simulink model "SolarPanelValidation"  (R2025a)
settings: Solver=VariableStepAuto  StartTime=0.0  StopTime=1.1*Voc/1  FixedStep=Ts  MaxStep=1e-3  RelTol=1e-3
PreLoadFcn:
  | % Parameterize the panel
  | SolarPanelValidationInput;
  | 
  | % Set the default test condition
  | irradiance = 1000;
  | temperature = 25;
values from neighbouring files (symbols this model uses):
  Isc = 8.18    [SolarPanelValidationInput.m]
  Np_cell = 3    [SolarPanelValidationInput.m]
  Ns_cell = 60    [SolarPanelValidationInput.m]
  Voc = 36.7    [SolarPanelValidationInput.m]
libraries: fl_lib x3, nesl_utility x3, ee_lib x1, simulink x1
CloseFcn:
  | try,close(h1_SolarPanelValidation),end
  | clear h1_SolarPanelValidation
  | 
  | clear CellTemperature  MaximumVoltage    TXIS1  irradianceVec
  | clear Irad NQ Tct  simlog_SolarPanelValidation
  | clear Isc Np_cell Tmeas  temperature
  | clear MaxP Ns_cell Voc  temperatureVec
  | clear MaximumCurrent  tout
  | clear MaximumPower  Rs   irradiance PanelIrradiance
Description:
  | Solar Panel Parameterization Validation
settings Model: Creator=The MathWorks, Inc.  LastModifiedBy=The MathWorks, Inc.
settings SolverCC: InitialStep=1e-3  AlgebraicLoopSolver=TrustRegion
settings DataIOCC: ReturnWorkspaceOutputs=off  OutputOption=SpecifiedOutputTimes  OutputTimes=[0:1.1*Voc/(1*1300):1.1*Voc/1]
settings OptimizationCC: ReuseModelBlockBuffer=off
settings DebuggingCC: UnconnectedInputMsg=warning  UnconnectedOutputMsg=warning  UnconnectedLineMsg=warning  StateNameClashWarn=warning  ArithmeticOperatorsInVariantConditions=warning
settings HardwareCC: ProdBitPerPointer=32.0  ProdBitPerSizeT=32.0  ProdBitPerPtrDiffT=32.0  ProdWordSize=32.0  ProdHWDeviceType=Intel->x86-32 (Windows32)
settings ModelReferenceCC: EnableRefExpFcnMdlSchedulingChecks=on  PropagateSignalLabelsOutOfModel=off
settings SFSimCC: CustomCodeUndefinedFunction=UseInterfaceOnly
settings RTWCC: GPUComputeCapability=3.5  DLArmComputeVersion=19.05
settings CodeAppCC: StateflowObjectComments=on
settings SimscapeCC: SimscapeLogType=all  SimscapeLogSimulationStatistics=on  SimscapeLogName=simlog_SolarPanelValidation

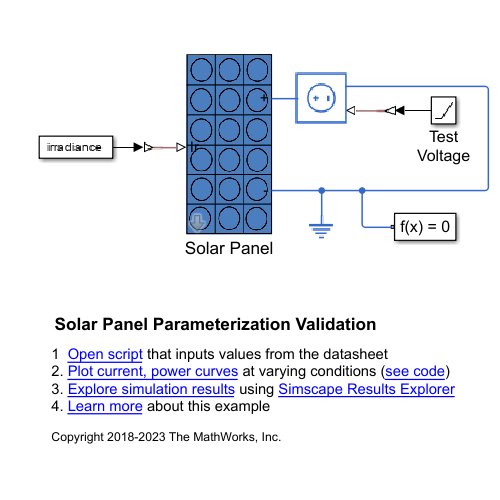
[thumbnail: Simulink's stored preview of the top-level diagram]
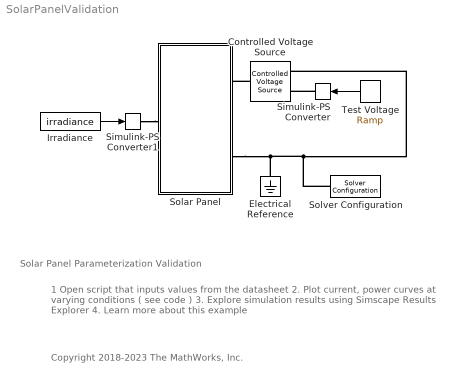
== system SolarPanelValidation ==
  note: Solar Panel Parameterization Validation
  note: 1 Open script that inputs values from the datasheet
      | 2. Plot current, power curves at varying conditions ( see code )
      | 3. Explore simulation results using Simscape Results Explorer
      | 4. Learn more about this example
  note: Copyright 2018-2023 The MathWorks, Inc.
  Controlled Voltage Source : fl_lib/Electrical/Electrical Sources/Controlled Voltage Source
  Electrical Reference : fl_lib/Electrical/Electrical Elements/Electrical Reference
  Irradiance : Constant  Value=irradiance
  Simulink-PS Converter : nesl_utility/Simulink-PS Converter  PhysicalDomain=network_engine_domain  SubClassName=ps_input  LeftPortType=input  RightPortType=output  PseudoPeriodic=off  Frequencies=[]  NoiseDistribution=none  NoiseParameters=[]  Unit=1  AffineConversion=off  FilteringAndDerivatives=provide  SimscapeFilterOrder=1  InputFilterTimeConstant=0.001  UdotUserProvided=0
  Simulink-PS Converter1 : nesl_utility/Simulink-PS Converter  PhysicalDomain=network_engine_domain  SubClassName=ps_input  LeftPortType=input  RightPortType=output  PseudoPeriodic=off  Frequencies=[]  NoiseDistribution=none  NoiseParameters=[]  Unit=1  AffineConversion=off  FilteringAndDerivatives=provide  SimscapeFilterOrder=1  InputFilterTimeConstant=0.001  UdotUserProvided=0
  Solar Panel : Subsystem  mask(Solar Panel){}
      mask help: Models a solar panel using a parallel-connected string of solar cells. The solar cell strings are modeled using a single Solar Cell block from the Simscape(TM) Electrical(TM) Sources library.
      mask Display: image('SolarPanelValidationIcon.jpg')
  Solver Configuration : nesl_utility/Solver Configuration  PhysicalDomain=network_engine_domain  SubClassName=solver  LeftPortType=input  RightPortType=generic  Tones=[]  Harmonics=[]  SimulateNoise=off  Profile=off  UseLocalSampling=off  EnableSwitchedLinearOptims=on  FrequencyDomain=off  UseCCode=off  RelTol=0.001  AbsTol=1e-06  MinStep=1e-09  ToWorkspace=off  RevertToSquareIcSolve=off  NumHomotopyIterations=100  PhasorMode=off  PhasorModeNumHarmonics=1  ConsistencySolver=NEWTON_FTOL  IndexReductionMethod=DerivativeReplacement  DoDC=off  ResidualTolerance=1e-09  ConsistencyTolSource=GLOBAL  ConsistencyAbsTol=0.001  ConsistencyRelTol=0.001  ConsistencyTolFactor=0.001  UseLocalSolver=off  LocalSolverChoice=NE_BACKWARD_EULER_ADVANCER  ResolveIndetEquations=on  FunctionEvalNumThread=1  LocalSolverSampleTime=1e-4  DoFixedCost=off  MaxNonlinIter=3  MaxModeIter=2  ComputeImpulses=off  ImpulseIterations=1  LinearAlgebra=auto  LinearAlgebraNumThread=0  EquationFormulation=NE_TIME_EF  DelaysMemoryBudget=1024  AutomaticFiltering=on  FilteringTimeConstant=0.001  PartitionStorageMethod=AS_NEEDED  PartitionMemoryBudget=1024  PartitionMethod=ROBUST  MultibodyUseLocalSolver=off  MultibodyLocalSolverChoice=ODE1  MultibodyLocalSolverSampleTime=0.001
  Test Voltage : simulink/Sources/Ramp  slope=1  start=0  InitialOutput=0
  wires:
  Irradiance/1 -> Simulink-PS Converter1/1
  Test Voltage/1 -> Simulink-PS Converter/1
  connections:
  Solver Configuration/RConn1 -- Controlled Voltage Source/RConn2 -- Electrical Reference/LConn1 -- Solar Panel/RConn2
  Controlled Voltage Source/LConn1 -- Solar Panel/RConn1
  Simulink-PS Converter/RConn1 -- Controlled Voltage Source/RConn1
  Simulink-PS Converter1/RConn1 -- Solar Panel/LConn1

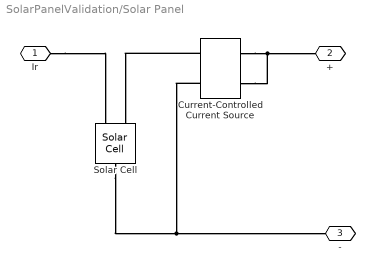
== system SolarPanelValidation/Solar Panel ==
  Current-Controlled Current Source : fl_lib/Electrical/Electrical Sources/Current-Controlled Current Source  K=-1*(Np_cell-1)  i1_specify=off  i1_priority=None  i1=0 A  i1_nominal_specify=off  i1_nominal_value=1  i1_nominal_unit=A  i2_specify=off  i2_priority=None  i2=0 A  i2_nominal_specify=off  i2_nominal_value=1  i2_nominal_unit=A
      settings: InternalSimscapePortConfiguration="{\"Bottom\":[],\"Left\":[{\"id\":\"p1\",\"label\":\"+\",\"type\":\"foundation.electrical.electrical\"},{\"id\":\"head\",\"label\":\"\",\"type\":\"foundation.electrical.electrical\"}],\"Right\":[{\"id\":\"n1\",\"label\":\"-\",\"type\":\"foundation.electrical.electrical\"},{\"id\":\"tail\",\"label\":\"\",\"type\":\"foundation.electrical.electrical\"}],\"Top\":[]}"
  Solar Cell : ee_lib/Sources/Solar Cell  prm=1  Isc=Isc/Np_cell A  Voc=Voc/Ns_cell V  Is=1e-6 A  Is2=0 A  Iph=7.34 A  Ir0=Irad W/m^2  ec=NQ  N2=2  Rs=Rs Ohm  Rp=inf Ohm  N_series=Ns_cell  N_parallel=1  TIPH1=Tct 1/K  EG=1.11 eV  TXIS1=TXIS1  TXIS2=3  TRS1=0  TRP1=0  Tmeas=Tmeas degC  TFIXED=temperature degC  thermal_mass=100 J/K  initial_temperature=25 degC
  Ir : PMIOPort  Side=Left
  + : PMIOPort  Port=2  Side=Right
  - : PMIOPort  Port=3  Side=Right
  connections:
  Current-Controlled Current Source/LConn2 -- -/RConn1 -- Solar Cell/RConn1
  Ir/RConn1 -- Solar Cell/LConn1
  Current-Controlled Current Source/LConn1 -- Solar Cell/LConn2
  Current-Controlled Current Source/RConn1 -- Current-Controlled Current Source/RConn2 -- +/RConn1
